simulink model "sistema1"  (R2025a)
settings: Solver=ode45  StartTime=0.0  StopTime=10.0  MaxStep=1e-2  RelTol=1e-3
settings Model: Creator=fabri  LastModifiedBy=fabri

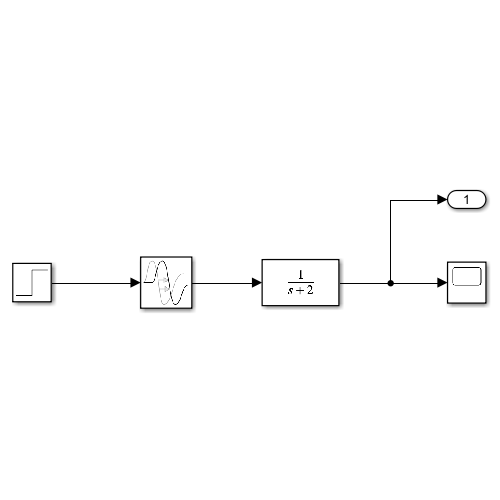
[thumbnail: Simulink's stored preview of the top-level diagram]
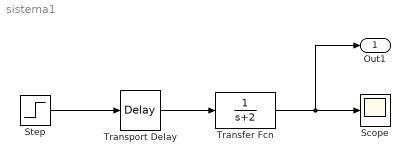
== system sistema1 ==
  Scope : Scope
      settings: ActiveDisplayYMinimum=-0.10295688803138847  ActiveDisplayYMaximum=0.60135216761380328
  Step : Step  Time=0  SampleTime=0
  Transfer Fcn : TransferFcn  Denominator=[1 2]
  Transport Delay : TransportDelay  DelayTime=5
  Out1 : Outport
  wires:
  Step/1 -> Transport Delay/1
  Transport Delay/1 -> Transfer Fcn/1
  Transfer Fcn/1 -> Out1/1, Scope/1
